simulink model "hydro"  (R2025a)
settings: Solver=VariableStepAuto  StartTime=0.0  StopTime=10.0  RelTol=1e-3
libraries: simulink x1
settings Model: Creator=Rishitha  LastModifiedBy=Rishitha

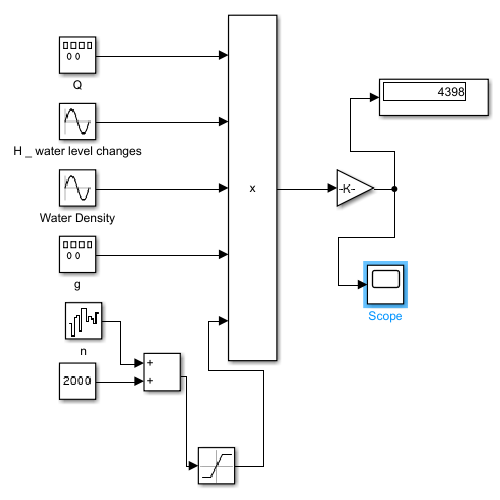
[thumbnail: Simulink's stored preview of the top-level diagram]
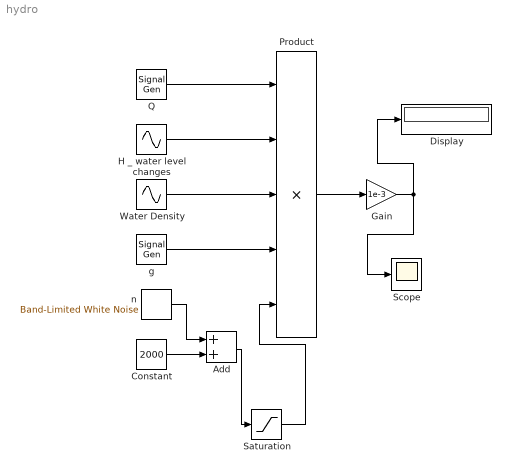
== system hydro ==
  Add : Sum
  Constant : Constant  Value=2000
  Display : Display
  Gain : Gain  Gain=1e-3
  H _ water level changes : Sin  Amplitude=50  Bias=100  Frequency=0.05  SampleTime=0
  Product : Product  Inputs=5
  Q : SignalGenerator  Amplitude=50  Frequency=0.1  Units=rad/sec
  Saturation : Saturate  UpperLimit=0.95  LowerLimit=0.75
  Scope : Scope
      settings: ActiveDisplayYMinimum=-649.76238886931628  ActiveDisplayYMaximum=6558.1816284088209
  Water Density : Sin  Amplitude=50  Bias=1500  Frequency=0.02  SampleTime=0
  "g " : SignalGenerator  Frequency=0.01
  n : simulink/Sources/Band-Limited White Noise  Cov=0.005  Ts=0.1  seed=[23341]
  wires:
  Saturation/1 -> Product/5
  Product/1 -> Gain/1
  Water Density/1 -> Product/3
  Add/1 -> Saturation/1
  Gain/1 -> Scope/1, Display/1
  Constant/1 -> Add/2
  "g "/1 -> Product/4
  Q/1 -> Product/1
  n/1 -> Add/1
  H _ water level changes/1 -> Product/2
